simulink model "AMF_model"  (R2026b)
settings: Solver=ode1  StopTime=0.01  FixedStep=Ts
PreLoadFcn:
  | ISC_Parameters
undefined symbols (not defined in the file): gamma0, gamma1, kappa, lambda, R, sigma0, Vc, Vd
settings Model: Creator=jeremiekemoun  LastModifiedBy=jeremiekemoun

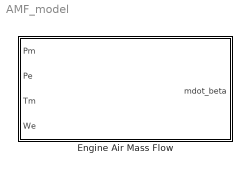
== system AMF_model ==
  Engine Air Mass Flow : Subsystem

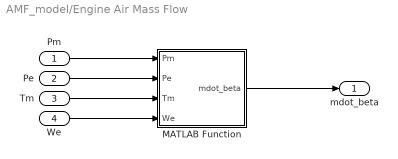
== system AMF_model/Engine Air Mass Flow ==
  Pm : Inport
  Pe : Inport  Port=2
  Tm : Inport  Port=3
  We : Inport  Port=4
  MATLAB Function : MATLAB Function  TreatAsAtomicUnit=on
  mdot_beta : Outport
  wires:
  Pe/1 -> MATLAB Function/2(Pe)
  Tm/1 -> MATLAB Function/3(Tm)
  We/1 -> MATLAB Function/4(We)
  MATLAB Function/1(mdot_beta) -> mdot_beta/1
  Pm/1 -> MATLAB Function/1(Pm)

== matlab function AMF_model/Engine Air Mass Flow/MATLAB Function ==
  data: Pm input; mdot_beta output; Pe input; Tm input; We input; R parameter; Vd parameter; Vc parameter; sigma0 parameter; kappa parameter; lambda parameter; gamma0 parameter; gamma1 parameter
function mdot_beta = fcn(Pm, Pe, Tm, We, R, Vd, Vc, sigma0, kappa, lambda, gamma0, gamma1)
% Engine Air Mass Flow: air mass flow leaving the intake manifold [kg/s]
% Inputs: Pm [Pa], Pe [Pa], Tm [K], We [rad/s]

% volumetric efficiency, pressure part (residual gas, polytropic expansion)
lam_lp = (Vc + Vd)/Vd - (Vc/Vd) * (Pe/Pm)^(1/kappa);

% volumetric efficiency, speed part (linear in We, identified in milestone 2)
lam_lw = gamma0 + gamma1*We;

% air mass flow into the engine (four-stroke engine: factor 1/2)
mdot_e = 0.5 * Pm/(R*Tm) * (lam_lp*lam_lw) * Vd * We/(2*pi);

% air mass flow from the manifold (the rest is fuel, ratio lambda*sigma0)
mdot_beta = mdot_e / (1 + 1/(lambda*sigma0));
